simulink model "hydel"  (R2025a)
settings: Solver=VariableStepAuto  StartTime=0.0  StopTime=10  RelTol=1e-3
libraries: spsRMSLib x2, spsThreePhaseParallelRLCLoadLib x1, spsLoadFlowBusLib x1, spsPowerLib x1, spsPower3phInstantaneousLib x1, spsExcitationSystemLib x1, spsHydraulicTurbineandGovernorLib x1, spsSynchronousMachinepuStandardLib x1, spsThreePhaseVIMeasurementLib x1, sps_lib x1
settings Model: Creator=Ram  LastModifiedBy=adhit

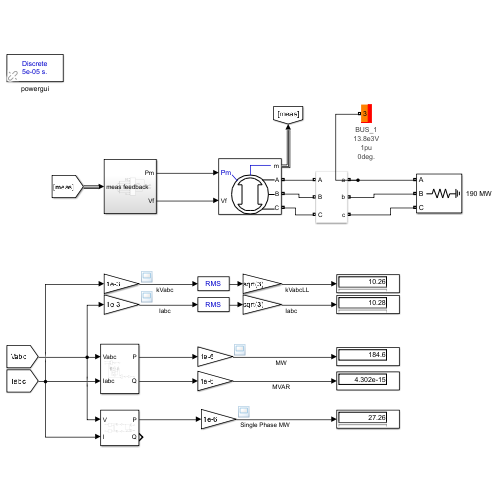
[thumbnail: Simulink's stored preview of the top-level diagram]
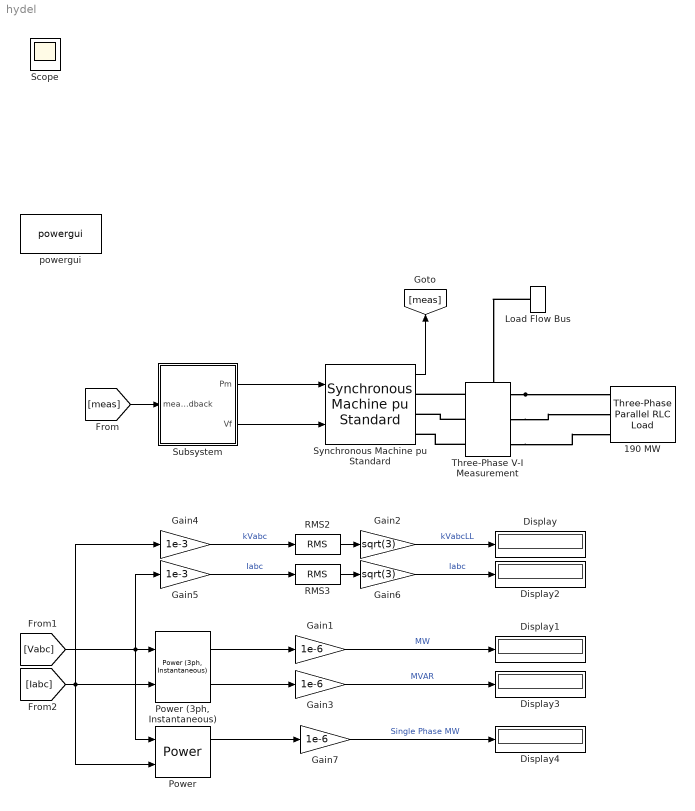
== system hydel ==
  190 MW : spsThreePhaseParallelRLCLoadLib/Three-Phase Parallel RLC Load  LConnTagsString=A|B|C  Configuration=Y (grounded)  NominalVoltage=(13800)*1  Vabc=[1e3 1e3 1e3]  Vabcp=[1e3 1e3 1e3]  NominalFrequency=50  UnbalancedPower=off  ActivePower=190000000  InductivePower=0  CapacitivePower=0  Pabc=[10e3 9e3 11e3]  QLabc=[100 90 110]  QCabc=[100 90 110]  Pabcp=[10e3 9e3 11e3]  QLabcp=[100 90 110]  QCabcp=[100 90 110]  Measurements=None  LoadType=constant PQ
  Display{,1..4} (5 alike) : Display
  Gain1 : Gain  Gain=1e-6
  Gain2 : Gain  Gain=sqrt(3)
  Gain3 : Gain  Gain=1e-6
  Gain4 : Gain  Gain=1e-3
  Gain5 : Gain  Gain=1e-3
  Gain6 : Gain  Gain=sqrt(3)
  Gain7 : Gain  Gain=1e-6
  Load Flow Bus : spsLoadFlowBusLib/Load Flow Bus  LConnTagsString=a  Phases=single  Connectors=on one side  ID=BUS_1  Vbase=13.8e3  Vref=1  Vangle=0  VLF=1  VLFb=1  VLFc=1  angleLF=0  angleLFb=0  angleLFc=0
  Power : spsPowerLib/Power  Freq=50  Vinit=[1, 0]  Iinit=[1, 0]  Ts=50e-6
  "Power (3ph, Instantaneous)" : spsPower3phInstantaneousLib/Power (3ph, Instantaneous)
  RMS2 : spsRMSLib/RMS  TrueRMS=on  Freq=60  RMSInit=120  Ts=0
  RMS3 : spsRMSLib/RMS  TrueRMS=on  Freq=60  RMSInit=120  Ts=0
  Subsystem : Subsystem
  Synchronous Machine pu Standard : spsSynchronousMachinepuStandardLib/Synchronous Machine pu Standard  PresetModel=No  MechanicalLoad=Mechanical power Pm  ShowDetailedParameters=on  RotorType=Salient-pole  Units=per unit standard parameters  MeasurementBus=off  NominalParameters=[190e6 13.8e3 50]  Reactances1=[ 1.81, 0.3, 0.23, 1.76, 0.65, 0.25, 0.15 ]  Reactances2=[2.24 0.17 0.12 1.02 0.13 0.08]  dAxisTimeConstants=Short-circuit  qAxisTimeConstants=Short-circuit  TimeConstants1="[ 4.4849  0.0681  0.1  ]"  TimeConstants2=[ 8.0, 0.03, 1.0, 0.07 ]  TimeConstants3="[  4.49  0.0681  0.0513  ]"  TimeConstants4=[ 8.0, 0.03, 0.3371, 0.0295 ]  TimeConstants5=[ 1.01, 0.053, 0.1 ]  TimeConstants6=[ 1.3201, 0.023, 1.0, 0.07 ]  TimeConstants7=[0.012 0.003 0.003]  TimeConstants8=[ 1.3201, 0.0231, 0.3371, 0.0295 ]  StatorResistance=0.037875  Mechanical=[0.1078 0.02056 8]  PolePairs=20  InitialConditions=[0 -45.4977 1 1 1 0 -120 120 2.31034]  SetSaturation=on  Saturation=[0.6404,0.7127,0.8441,0.9214,0.9956,1.082,1.19,1.316,1.457;0.7,0.7698,0.8872,0.9466,0.9969,1.046,1.1,1.151,1.201]  LoadFlowParameters=[1,0,0,0,0]  TsPowergui=0  TsBlock=50e-6  IterativeModel=Trapezoidal non iterative  IterativeDiscreteModel=Trapezoidal non iterative  BusType=swing  Pref=0  Qref=0  Qmin=-Inf  Qmax=Inf  PLF=0  QLF=0
  Three-Phase V-I Measurement : spsThreePhaseVIMeasurementLib/Three-Phase V-I Measurement  VoltageMeasurement=phase-to-ground  SetLabelV=on  LabelV=Vabc  Vpu=off  VpuLL=off  CurrentMeasurement=yes  SetLabelI=on  LabelI=Iabc  Ipu=off  Pbase=100e6  Vbase=500e3  OutputType=Complex  PhasorSimulation=off  PSBequivalent=0
  powergui : sps_lib/powergui  Priority=1  SimulationMode=Discrete  SampleTime=50e-6  frequency=60  Iterations=50  frequencyindice=50  Pbase=100e6  ErrMax=1e-4  UnitsV=kV  UnitsW=MW  buscounter=0  FunctionMessages=off  echomessages=off  EnableUseOfTLC=off  CurrentSourceSwitches=off  DisableSnubberDevices=off  DisableRonSwitches=off  DisableVfSwitches=off  DisplayEquations=off  AutomaticDiscreteSolvers=off  SolverType=Tustin/Backward Euler (TBE)  Interpol=off  ExternalGateDelay=off  methode=off  Ts=100  x0status=blocks  SPID=on  SwTol=0  HookPort=off  NonlinearTolerance=1e-4  nMaxIteration=100  ContinueOnMaxIteration=off  RestoreLinks=warning  ResistiveCurrentMeasurement=off  Frange=[0:2:500]  Ylog=off  Xlog=on  ShowGrid=off  save=off  variable=ZData  structure=0  ZoomFFT=off  StartTime=0.0  cycles=1  DisplayStyle=1  fundamental=60  FreqAxis=off  MaxFrequency=1000  frequencyindicesteady=1  RmsSteady=1  display=off
  Scope : Scope
      settings: ActiveDisplayYMinimum=-31.413971084134396  ActiveDisplayYMaximum=33.099589831706609
  wires:
  Synchronous Machine pu Standard/1 -> [meas]
  [meas] -> Subsystem/1(meas feedback)
  Subsystem/1(Pm) -> Synchronous Machine pu Standard/1
  Subsystem/2(Vf) -> Synchronous Machine pu Standard/2
  [Vabc] -> Power/1, "Power (3ph, Instantaneous)"/1, Gain5/1
  [Iabc] -> Power/2, Gain4/1, "Power (3ph, Instantaneous)"/2
  Gain4/1 -> RMS2/1  "kVabc"
  "Power (3ph, Instantaneous)"/1 -> Gain1/1
  Gain1/1 -> Display1/1  "MW"
  "Power (3ph, Instantaneous)"/2 -> Gain3/1
  Gain3/1 -> Display3/1  "MVAR"
  Gain5/1 -> RMS3/1  "Iabc"
  RMS2/1 -> Gain2/1
  Gain2/1 -> Display/1  "kVabcLL"
  Gain6/1 -> Display2/1  "Iabc"
  RMS3/1 -> Gain6/1
  Power/1 -> Gain7/1
  Gain7/1 -> Display4/1  "Single Phase MW"
  connections:
  Three-Phase V-I Measurement/LConn1 -- Synchronous Machine pu Standard/RConn1
  Three-Phase V-I Measurement/LConn2 -- Synchronous Machine pu Standard/RConn2
  Three-Phase V-I Measurement/LConn3 -- Synchronous Machine pu Standard/RConn3
  Three-Phase V-I Measurement/RConn1 -- Load Flow Bus/LConn1 -- 190 MW/LConn1
  Three-Phase V-I Measurement/RConn2 -- 190 MW/LConn2
  Three-Phase V-I Measurement/RConn3 -- 190 MW/LConn3

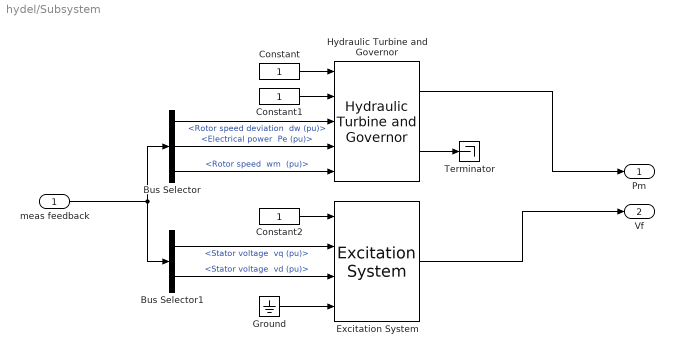
== system hydel/Subsystem ==
  meas feedback : Inport
  Bus Selector : BusSelector  OutputSignals="Mechanical.Rotor speed deviation  dw (pu),Mechanical.Electrical power  Pe (pu),Mechanical.Rotor speed  wm  (pu)"
  Bus Selector1 : BusSelector  OutputSignals="dq0 components.Stator voltage  vq (pu),dq0 components.Stator voltage  vd (pu)"
  Constant : Constant
  Constant1 : Constant
  Constant2 : Constant
  Excitation System : spsExcitationSystemLib/Excitation System  tr=20e-3  reg=[ 300, 0.001 ]  exc=[ 1, 0 ]  tgr=[ 0, 0 ]  damp=[ 0.01, 0.1 ]  sat=[ 0, 0 ]  lim=[ -11.5, 11.5, 0 ]  v0=[1 2.3103]
      settings: LibrarySourceBlock=sps_lib/Electrical Machines/Synchronous Machine Control/Excitation System
  Ground : Ground
  Hydraulic Turbine and Governor : spsHydraulicTurbineandGovernorLib/Hydraulic Turbine and Governor  sm="[ 10/3  0.07 ]"  gate="[  0.01  0.97518  -0.1  0.1 ]"  reg="[  0.05  1  0.2  0.1  0.01  ]"  hyd="[  0  2.67  ]"  dref=0  po=1.0094
      settings: LibrarySourceBlock=|
      | sps_lib/Electrical Machines/Synchronous Machine Control/Hydraulic Turbine
      | and Governor
  Terminator : Terminator
  Pm : Outport
  Vf : Outport  Port=2
  wires:
  meas feedback/1 -> Bus Selector/1, Bus Selector1/1
  Bus Selector1/2 -> Excitation System/3  "<Stator voltage  vd (pu)>"
  Constant2/1 -> Excitation System/1
  Bus Selector1/1 -> Excitation System/2  "<Stator voltage  vq (pu)>"
  Excitation System/1 -> Vf/1
  Ground/1 -> Excitation System/4
  Hydraulic Turbine and Governor/2 -> Terminator/1
  Hydraulic Turbine and Governor/1 -> Pm/1
  Constant/1 -> Hydraulic Turbine and Governor/1
  Bus Selector/1 -> Hydraulic Turbine and Governor/3  "<Rotor speed deviation  dw (pu)>"
  Constant1/1 -> Hydraulic Turbine and Governor/2
  Bus Selector/2 -> Hydraulic Turbine and Governor/4  "<Electrical power  Pe (pu)>"
  Bus Selector/3 -> Hydraulic Turbine and Governor/5  "<Rotor speed  wm  (pu)>"
